simulink model "ace_cl_virtual"  (R2026a)
settings: Solver=ode23tb  StopTime=C.cl_T  MaxStep=1e-3
PreLoadFcn:
  | ace_params;
InitFcn:
  | ace_params;
values from neighbouring files (symbols this model uses):
  C = struct()    [ace_params.m]    (also in build_ace_sysid_pipeline.m = evalin('base', 'C'))
libraries: slpidlib x1
settings Model: Creator=00782620  LastModifiedBy=00782620

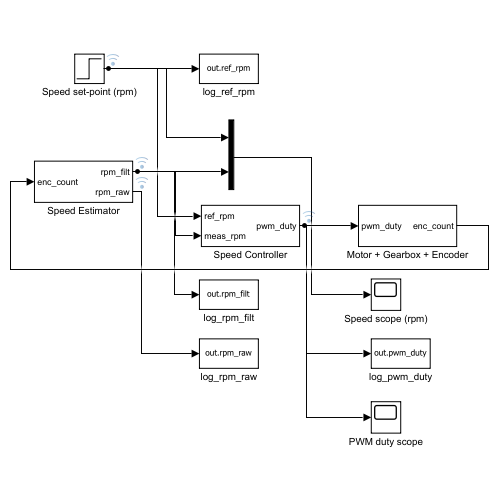
[thumbnail: Simulink's stored preview of the top-level diagram]
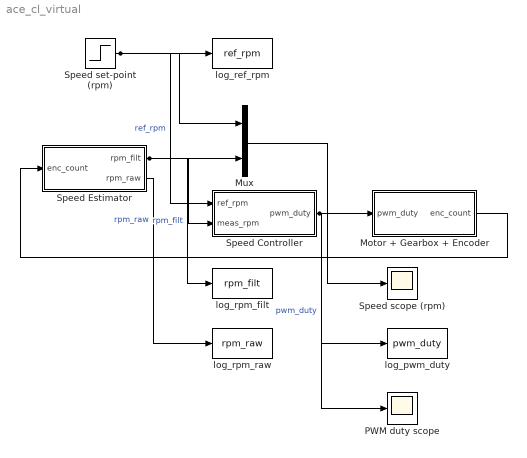
== system ace_cl_virtual ==
  Motor + Gearbox + Encoder : Subsystem
  Mux : Mux  Inputs=2
  PWM duty scope : Scope
  Speed Controller : Subsystem
  Speed Estimator : Subsystem
  Speed scope (rpm) : Scope
  Speed set-point (rpm) : Step  Time=C.t_step_hw  FinalValue=C.ref_rpm  SampleTime=C.Ts
  log_pwm_duty : ToWorkspace  VariableName=pwm_duty  SaveFormat=Timeseries  SampleTime=-1
  log_ref_rpm : ToWorkspace  VariableName=ref_rpm  SaveFormat=Timeseries  SampleTime=-1
  log_rpm_filt : ToWorkspace  VariableName=rpm_filt  SaveFormat=Timeseries  SampleTime=-1
  log_rpm_raw : ToWorkspace  VariableName=rpm_raw  SaveFormat=Timeseries  SampleTime=-1
  wires:
  Motor + Gearbox + Encoder/1(enc_count) -> Speed Estimator/1(enc_count)
  Mux/1 -> Speed scope (rpm)/1
  Speed set-point (rpm)/1 -> Speed Controller/1(ref_rpm), log_ref_rpm/1, Mux/1  "ref_rpm"
  Speed Estimator/1(rpm_filt) -> Speed Controller/2(meas_rpm), log_rpm_filt/1, Mux/2  "rpm_filt"
  Speed Controller/1(pwm_duty) -> Motor + Gearbox + Encoder/1(pwm_duty), PWM duty scope/1, log_pwm_duty/1  "pwm_duty"
  Speed Estimator/2(rpm_raw) -> log_rpm_raw/1  "rpm_raw"

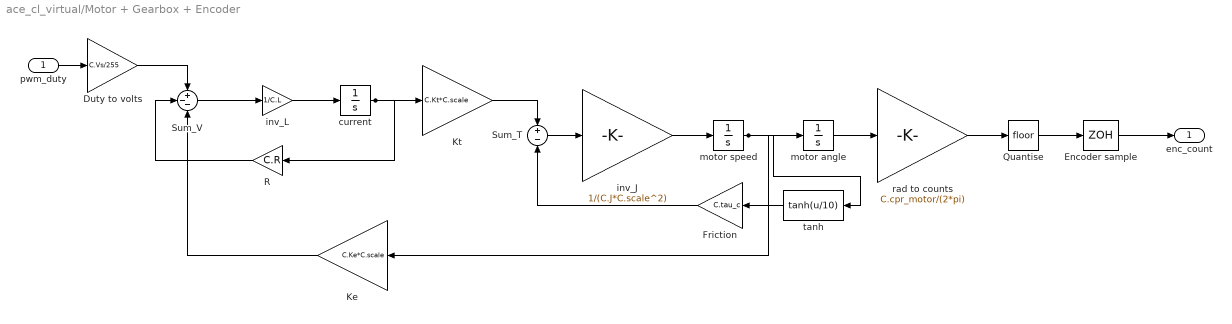
== system ace_cl_virtual/Motor + Gearbox + Encoder ==
  pwm_duty : Inport
  Duty to volts : Gain  Gain=C.Vs/255
  Encoder sample : ZeroOrderHold  SampleTime=C.Ts
  Friction : Gain  Gain=C.tau_c
  Ke : Gain  Gain=C.Ke*C.scale
  Kt : Gain  Gain=C.Kt*C.scale
  Quantise : Rounding
  R : Gain  Gain=C.R
  Sum_T : Sum  Inputs=+-
  Sum_V : Sum  Inputs=+--
  current : Integrator
  inv_J : Gain  Gain=1/(C.J*C.scale^2)
  inv_L : Gain  Gain=1/C.L
  motor angle : Integrator
  motor speed : Integrator
  rad to counts : Gain  Gain=C.cpr_motor/(2*pi)
  tanh : Fcn  Expr=tanh(u/10)
  enc_count : Outport
  wires:
  pwm_duty/1 -> Duty to volts/1
  R/1 -> Sum_V/2
  Kt/1 -> Sum_T/1
  inv_L/1 -> current/1
  Duty to volts/1 -> Sum_V/1
  Ke/1 -> Sum_V/3
  Sum_V/1 -> inv_L/1
  current/1 -> R/1, Kt/1
  Sum_T/1 -> inv_J/1
  inv_J/1 -> motor speed/1
  Friction/1 -> Sum_T/2
  motor speed/1 -> Ke/1, tanh/1, motor angle/1
  tanh/1 -> Friction/1
  motor angle/1 -> rad to counts/1
  rad to counts/1 -> Quantise/1
  Quantise/1 -> Encoder sample/1
  Encoder sample/1 -> enc_count/1

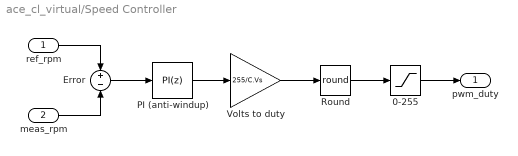
== system ace_cl_virtual/Speed Controller ==
  ref_rpm : Inport
  meas_rpm : Inport  Port=2
  0-255 : Saturate  UpperLimit=255  LowerLimit=0
  Error : Sum  Inputs=+-
  PI (anti-windup) : slpidlib/PID Controller  Controller=PI  Form=Parallel  TimeDomain=Discrete-time  UseExternalTs=off  SampleTime=C.Ts  IntegratorMethod=Forward Euler  FilterMethod=Forward Euler  ControllerParametersSource=internal  P=C.Kp  I=C.Ki  UseKiTs=off  D=0  UseExternalDerivativeSource=off  N=100  UseFilter=on  TunerSelectOption=Transfer Function Based (PID Tuner App)  InitialConditionSource=internal  InitialConditionForIntegrator=0  InitialConditionForFilter=0  DifferentiatorICPrevScaledInput=0  ExternalReset=none  TrackingMode=off  Kt=1  LimitOutput=on  SatLimitsSource=internal  UpperSaturationLimit=C.Vs  LowerSaturationLimit=0  LinearizeAsGain=off  AntiWindupMode=clamping  Kb=1  LimitIntegrator=off  UpperIntegratorSaturationLimit=inf  LowerIntegratorSaturationLimit=-inf  POutMin=[]  POutMax=[]  IOutMin=[]  IOutMax=[]  DOutMin=[]  DOutMax=[]  NOutMin=[]  NOutMax=[]  SumOutMin=[]  SumOutMax=[]  SaturationOutMin=[]  SaturationOutMax=[]  PParamMin=[]  PParamMax=[]  IParamMin=[]  IParamMax=[]  DParamMin=[]  DParamMax=[]  NParamMin=[]  NParamMax=[]  KbParamMin=[]  KbParamMax=[]  KtParamMin=[]  KtParamMax=[]  KbOutMin=[]  KbOutMax=[]  KtOutMin=[]  KtOutMax=[]  IntegratorOutMin=[]  IntegratorOutMax=[]  FilterOutMin=[]  FilterOutMax=[]  SumI1OutMin=[]  SumI1OutMax=[]  SumI2OutMin=[]  SumI2OutMax=[]  SumI3OutMin=[]  SumI3OutMax=[]  SumI4OutMin=[]  SumI4OutMax=[]  SumDOutMin=[]  SumDOutMax=[]  DifferentiatorOutMin=[]  DifferentiatorOutMax=[]  FilterDiffOutCoefMin=[]  FilterDiffOutCoefMax=[]  ReciprocalOutMin=[]  ReciprocalOutMax=[]  SumDenOutMin=[]  SumDenOutMax=[]  SumNumOutMin=[]  SumNumOutMax=[]  DivideOutMin=[]  DivideOutMax=[]  UdiffTsProdOutMin=[]  UdiffTsProdOutMax=[]  NTsProdOutMin=[]  NTsProdOutMax=[]  UintegralTsProdOutMin=[]  UintegralTsProdOutMax=[]  UngainTsProdOutMin=[]  UngainTsProdOutMax=[]  ClampingZeroOutDataTypeStr=Inherit: Inherit via back propagation  ClampingZeroOutMin=[]  ClampingZeroOutMax=[]  FilterDenConstantOutDataTypeStr=Inherit: Inherit via back propagation  FilterDenConstantOutMin=[]  FilterDenConstantOutMax=[]  PCopyOutDataTypeStr=Inherit: Inherit via back propagation  PCopyOutMin=[]  PCopyOutMax=[]  NCopyOutDataTypeStr=Inherit: Inherit via back propagation  NCopyOutMin=[]  NCopyOutMax=[]  IntegratorContinuousStateAttributes=''  IntegratorStateMustResolveToSignalObject=off  IntegratorRTWStateStorageClass=Auto  FilterContinuousStateAttributes=''  FilterStateMustResolveToSignalObject=off  FilterRTWStateStorageClass=Auto  ParallelPVariant=InternalParameters  IdealPVariant=Disabled  IVariant=InternalParameters  DVariant=Disabled  IntegratorVariant=Discrete  SatVariant=Enabled  AWVariant=DiscClampingParallel  PCopyVariant=Disabled  TRVariant=Disabled  FdbkBlocksVariant=Forward  IdealPFdbkVariant=Disabled  SatFdbkVariant=Disabled  DerivativeFilterVariant=Disabled  NVariant=Disabled  NCopyVariant=Disabled_SignalSpec  FilterICVariant=Disabled  IntegratorICVariant=InternalICs  ExternalResetVariant=Disabled  TRSumVariant=Passthrough  SumFdbkVariant=Disabled  SumVariant=Sum_PI  TsampFilterVariant=InternalTs  TsampNgainVariant=Passthrough  TsampIntegralVariant=Disabled_SignalSpec  ExternalSaturationOutDataTypeStr=Inherit: Same as second input  DerivativeSourceVariant=Disabled  PreIntVariant=InternalPreInt
      settings: LibrarySourceBlock=simulink/Discrete/Discrete PID Controller
  Round : Rounding  Operator=round
  Volts to duty : Gain  Gain=255/C.Vs
  pwm_duty : Outport
  wires:
  Error/1 -> PI (anti-windup)/1
  ref_rpm/1 -> Error/1
  Volts to duty/1 -> Round/1
  meas_rpm/1 -> Error/2
  PI (anti-windup)/1 -> Volts to duty/1
  Round/1 -> 0-255/1
  0-255/1 -> pwm_duty/1

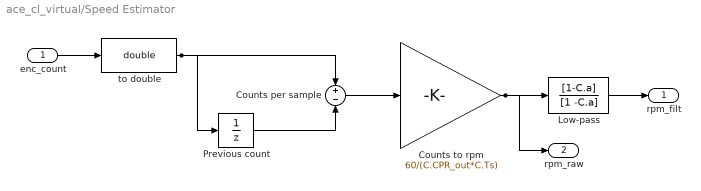
== system ace_cl_virtual/Speed Estimator ==
  enc_count : Inport
  Counts per sample : Sum  Inputs=+-
  Counts to rpm : Gain  Gain=60/(C.CPR_out*C.Ts)
  Low-pass : DiscreteTransferFcn  Numerator=[1-C.a]  Denominator=[1 -C.a]  SampleTime=C.Ts
  Previous count : UnitDelay  SampleTime=C.Ts
  to double : DataTypeConversion  OutDataTypeStr=double  SaturateOnIntegerOverflow=off  RndMeth=Floor
  rpm_filt : Outport
  rpm_raw : Outport  Port=2
  wires:
  Counts to rpm/1 -> Low-pass/1, rpm_raw/1
  Counts per sample/1 -> Counts to rpm/1
  Previous count/1 -> Counts per sample/2
  enc_count/1 -> to double/1
  to double/1 -> Counts per sample/1, Previous count/1
  Low-pass/1 -> rpm_filt/1
